simulink model "OFDM_Communication_Model_Start"  (R2024a)
settings: Solver=FixedStepDiscrete  StartTime=0.0  StopTime=0.2*4  RelTol=1e-3  EnableMultiTasking=on
model workspace: external: MAT-File modelspace.mat (data not in the file)
libraries: dspxfrm3 x3, commdigbbndpm3 x2, matrix_library x2
settings Model: Creator=thua3267  LastModifiedBy=hcha7553
settings SolverCC: AlgebraicLoopSolver=TrustRegion  AutoInsertRateTranBlk=on
settings DataIOCC: LimitDataPoints=on  ReturnWorkspaceOutputs=off
settings OptimizationCC: LifeSpan=inf
settings DebuggingCC: UnconnectedInputMsg=warning  UnconnectedOutputMsg=warning  UnconnectedLineMsg=warning  AllowSymbolicDim=off  SFUnexpectedBacktrackingDiag=warning  SFNoUnconditionalDefaultTransitionDiag=warning  SFExecutionAtInitializationDiag=none  ArithmeticOperatorsInVariantConditions=warning
settings ModelReferenceCC: EnableRefExpFcnMdlSchedulingChecks=on  PropagateSignalLabelsOutOfModel=off
settings SFSimCC: SimUseLocalCustomCode=off  CustomCodeUndefinedFunction=UseInterfaceOnly
settings RTWCC: RTWUseLocalCustomCode=off  GPUComputeCapability=3.5
settings CodeAppCC: StateflowObjectComments=on
settings GRTTargetCC: TargetLangStandard=C89/C90 (ANSI)
settings ConfigComp: CovMetricSettings=dw  CovSaveCumulativeToWorkspaceVar=on  CovSaveSingleToWorkspaceVar=on  CovExternalEMLEnable=off

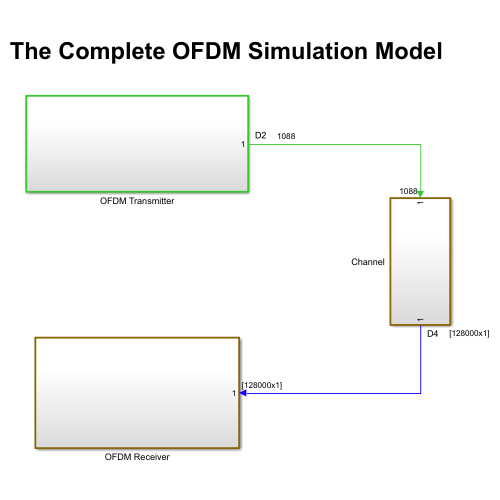
[thumbnail: Simulink's stored preview of the top-level diagram]
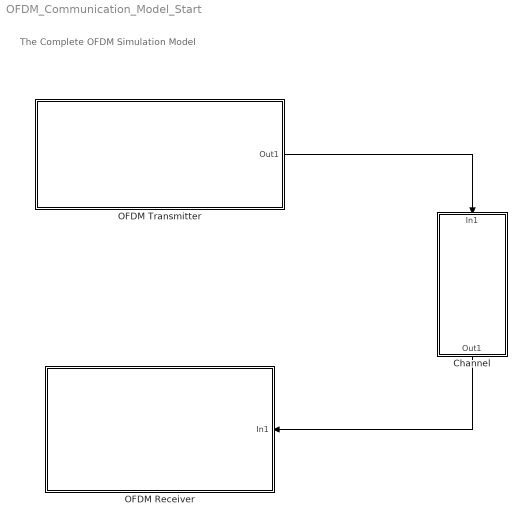
== system OFDM_Communication_Model_Start ==
  note: The Complete OFDM Simulation Model
  Channel : Subsystem
  OFDM Receiver : Subsystem
  OFDM Transmitter : Subsystem
  wires:
  OFDM Transmitter/1(Out1) -> Channel/1(In1)
  Channel/1(Out1) -> OFDM Receiver/1(In1)

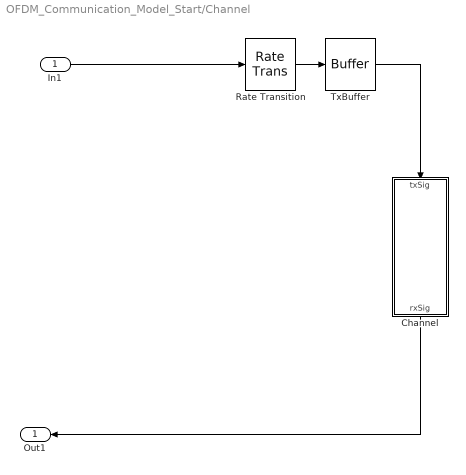
== system OFDM_Communication_Model_Start/Channel ==
  In1 : Inport
  Channel : MATLAB Function  TreatAsAtomicUnit=on
  Rate Transition : RateTransition  OutPortSampleTime=1/640e3*1280
  TxBuffer : Buffer  N=128000
  Out1 : Outport  VectorParamsAs1DForOutWhenUnconnected=off
  wires:
  In1/1 -> Rate Transition/1
  Channel/1(rxSig) -> Out1/1
  TxBuffer/1 -> Channel/1(txSig)
  Rate Transition/1 -> TxBuffer/1

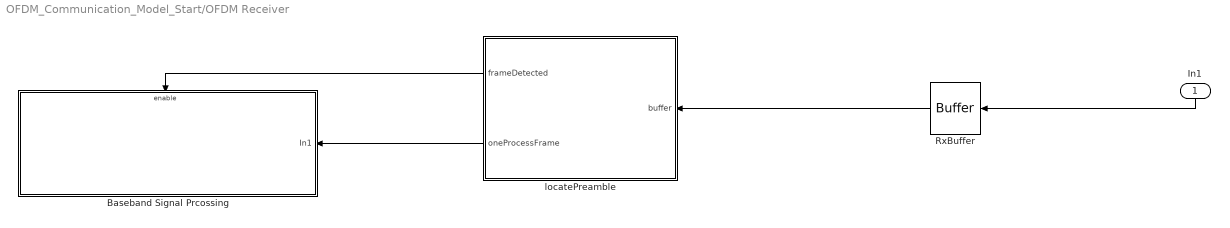
== system OFDM_Communication_Model_Start/OFDM Receiver ==
  In1 : Inport
  Baseband Signal Prcossing : Subsystem  TreatAsAtomicUnit=on
  RxBuffer : Buffer  N=1280*2  V=1280
  locatePreamble : MATLAB Function  TreatAsAtomicUnit=on
  wires:
  locatePreamble/2(oneProcessFrame) -> Baseband Signal Prcossing/1(In1)
  locatePreamble/1(frameDetected) -> Baseband Signal Prcossing/Enable
  In1/1 -> RxBuffer/1
  RxBuffer/1 -> locatePreamble/1(buffer)

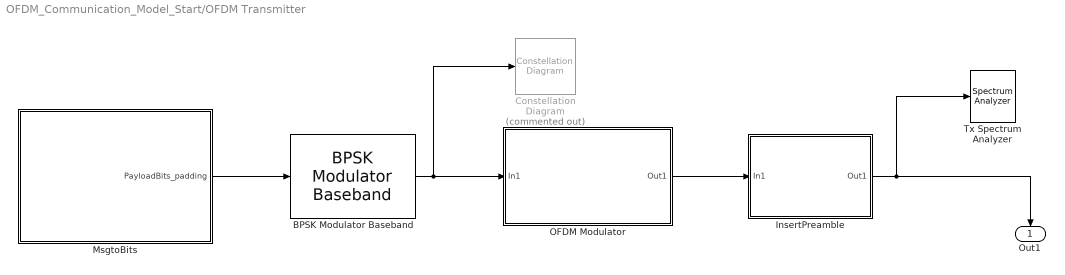
== system OFDM_Communication_Model_Start/OFDM Transmitter ==
  BPSK Modulator Baseband : commdigbbndpm3/BPSK Modulator Baseband  Ph=0  outDtype=double  outWordLen=16  outUDDataType=sfix(16)  outFracLenMode=Best precision  outFracLen=15  outDataTypeStr=double  outLastDataTypeStr=double
  Constellation Diagram : ConstellationDiagram  Commented=on  WindowPosition=[1 41 1920 964]  DefaultConfigurationName=comm.scopes.ConstellationDiagramBlockCfg
  InsertPreamble : Subsystem
  MsgtoBits : MATLAB Function  TreatAsAtomicUnit=on
  OFDM Modulator : Subsystem
  Tx Spectrum Analyzer : SpectrumAnalyzer  WindowPosition=[491.000000,211.000000,299.000000,298.000000,]  Visible=on  ScopeFrameLocation=window  Method=Welch  SampleRate=640000  Span=544000  StartFrequency=-272000  StopFrequency=272000  AveragingMethod=Running  YLimits=[-78.9896859,-0.36696175]  ColorLimits=[-29.698374910183748,-7.1171834026087382]  AllowFFTLengthLessThanSamplesPerUpdate=on  DefaultConfigurationName=spbscopes.SpectrumAnalyzerBlockCfg  IsFrequencyInputMode=0  FrequencyVectorPort=0  FrequencyVectorFromPort=0  FrequencyInputRBWPort=0  FrequencyInputRBWFromPort=0
  Out1 : Outport  VectorParamsAs1DForOutWhenUnconnected=off
  wires:
  MsgtoBits/1(PayloadBits_padding) -> BPSK Modulator Baseband/1
  InsertPreamble/1(Out1) -> Out1/1, Tx Spectrum Analyzer/1
  BPSK Modulator Baseband/1 -> Constellation Diagram/1, OFDM Modulator/1(In1)
  OFDM Modulator/1(Out1) -> InsertPreamble/1(In1)

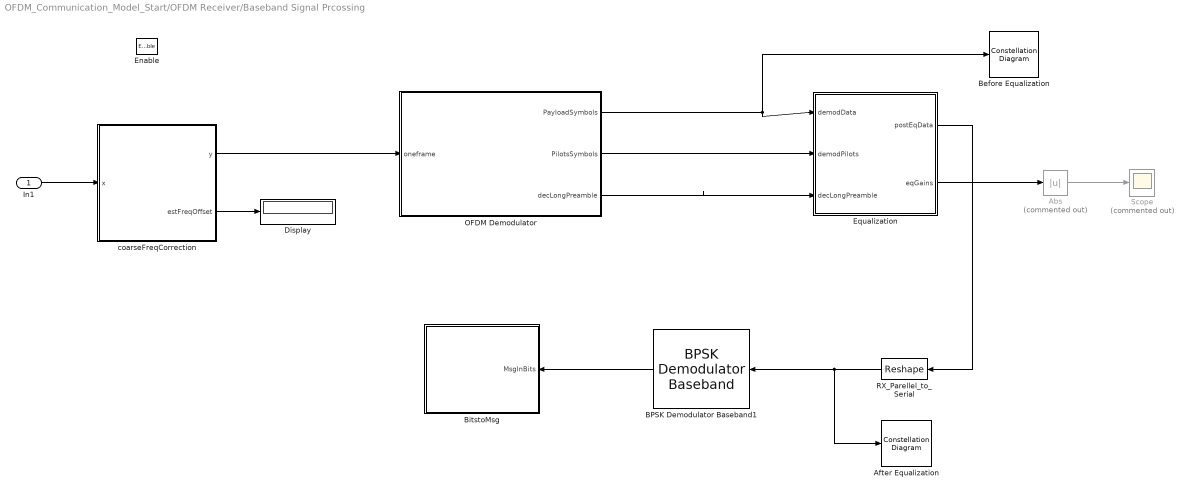
== system OFDM_Communication_Model_Start/OFDM Receiver/Baseband Signal Prcossing ==
  In1 : Inport
  Enable : EnablePort
  " Equalization" : MATLAB Function  TreatAsAtomicUnit=on
  " RX_Parellel_to_Serial" : Reshape  OutputDimensionality=Column vector (2-D)
  " coarseFreqCorrection" : MATLAB Function  TreatAsAtomicUnit=on
  Abs : Abs  Commented=on  SaturateOnIntegerOverflow=off
  After Equalization : ConstellationDiagram  WindowPosition=[486.000000,209.000000,309.000000,302.000000,]  Visible=on  ScopeFrameLocation=window  SymbolsToDisplay=12  ReferenceConstellation=BPSK  XLimits=[-4 4]  YLimits=[-4 4]  DefaultConfigurationName=comm.scopes.ConstellationDiagramBlockCfg
  BPSK Demodulator Baseband1 : commdigbbndpm3/BPSK Demodulator Baseband  DecType=Hard decision  VarSource=Dialog  Variance=1  Ph=0  outDtype=Inherit via internal rule  derotateFactorWordLen=16  derotateFactorDataTypeStr=Inherit: Same word length as input  derotateFactorLastDataTypeStr=Inherit: Same word length as input
  Before Equalization : ConstellationDiagram  WindowPosition=[474.000000,209.000000,332.000000,302.000000,]  Visible=on  ScopeFrameLocation=window  SymbolsToDisplay=1  ReferenceConstellation=BPSK  XLimits=[-0.039844 0.03808]  YLimits=[-0.043559 0.034365]  DefaultConfigurationName=comm.scopes.ConstellationDiagramBlockCfg
  BitstoMsg : MATLAB Function  TreatAsAtomicUnit=on
  Display : Display
  OFDM Demodulator : Subsystem
  Scope : Scope  Commented=on
  wires:
  In1/1 -> " coarseFreqCorrection"/1(x)
  " coarseFreqCorrection"/2(estFreqOffset) -> Display/1
  BPSK Demodulator Baseband1/1 -> BitstoMsg/1(MsgInBits)
  " Equalization"/1(postEqData) -> " RX_Parellel_to_Serial"/1
  " RX_Parellel_to_Serial"/1 -> After Equalization/1, BPSK Demodulator Baseband1/1
  " coarseFreqCorrection"/1(y) -> OFDM Demodulator/1(oneframe)
  " Equalization"/2(eqGains) -> Abs/1
  Abs/1 -> Scope/1
  OFDM Demodulator/1(PayloadSymbols) -> Before Equalization/1, " Equalization"/1(demodData)
  OFDM Demodulator/2(PilotsSymbols) -> " Equalization"/2(demodPilots)
  OFDM Demodulator/3(decLongPreamble) -> " Equalization"/3(decLongPreamble)

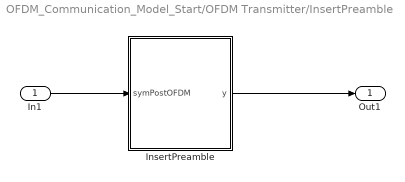
== system OFDM_Communication_Model_Start/OFDM Transmitter/InsertPreamble ==
  In1 : Inport
  InsertPreamble : MATLAB Function  TreatAsAtomicUnit=on
  Out1 : Outport  VectorParamsAs1DForOutWhenUnconnected=off
  wires:
  InsertPreamble/1(y) -> Out1/1
  In1/1 -> InsertPreamble/1(symPostOFDM)

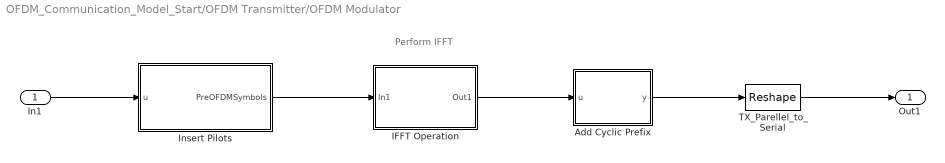
== system OFDM_Communication_Model_Start/OFDM Transmitter/OFDM Modulator ==
  note: Perform IFFT
  In1 : Inport
  " TX_Parellel_to_Serial" : Reshape  OutputDimensionality=Column vector (2-D)
  Add Cyclic Prefix : MATLAB Function  TreatAsAtomicUnit=on
  IFFT Operation : Subsystem
  Insert Pilots : MATLAB Function  TreatAsAtomicUnit=on
  Out1 : Outport  VectorParamsAs1DForOutWhenUnconnected=off
  wires:
  " TX_Parellel_to_Serial"/1 -> Out1/1
  Add Cyclic Prefix/1(y) -> " TX_Parellel_to_Serial"/1
  In1/1 -> Insert Pilots/1(u)
  Insert Pilots/1(PreOFDMSymbols) -> IFFT Operation/1(In1)
  IFFT Operation/1(Out1) -> Add Cyclic Prefix/1(u)

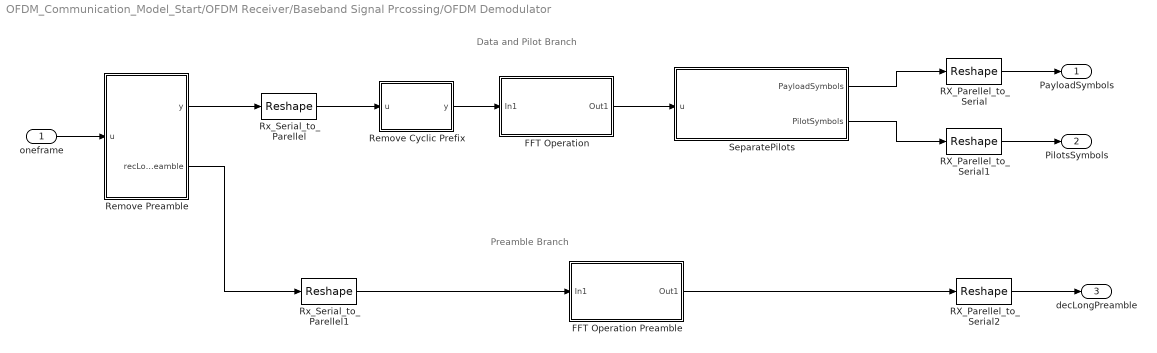
== system OFDM_Communication_Model_Start/OFDM Receiver/Baseband Signal Prcossing/OFDM Demodulator ==
  note: Data and Pilot Branch
  note: Preamble Branch
  oneframe : Inport
  " RX_Parellel_to_Serial" : Reshape  OutputDimensionality=Column vector (2-D)
  " RX_Parellel_to_Serial1" : Reshape  OutputDimensionality=Column vector (2-D)
  " RX_Parellel_to_Serial2" : Reshape  OutputDimensionality=Column vector (2-D)
  FFT Operation : Subsystem
  FFT Operation Preamble : Subsystem
  Remove Cyclic Prefix : MATLAB Function  TreatAsAtomicUnit=on
  "Remove Preamble " : MATLAB Function  TreatAsAtomicUnit=on
  Rx_Serial_to_Parellel : Reshape  OutputDimensionality=Customize  OutputDimensions=[80 12]
  Rx_Serial_to_Parellel1 : Reshape  OutputDimensionality=Customize  OutputDimensions=[64 2]
  SeparatePilots : MATLAB Function  TreatAsAtomicUnit=on
  PayloadSymbols : Outport  VectorParamsAs1DForOutWhenUnconnected=off
  PilotsSymbols : Outport  Port=2  VectorParamsAs1DForOutWhenUnconnected=off
  decLongPreamble : Outport  Port=3  VectorParamsAs1DForOutWhenUnconnected=off
  wires:
  " RX_Parellel_to_Serial"/1 -> PayloadSymbols/1
  Rx_Serial_to_Parellel/1 -> Remove Cyclic Prefix/1(u)
  Remove Cyclic Prefix/1(y) -> FFT Operation/1(In1)
  FFT Operation/1(Out1) -> SeparatePilots/1(u)
  SeparatePilots/1(PayloadSymbols) -> " RX_Parellel_to_Serial"/1
  "Remove Preamble "/1(y) -> Rx_Serial_to_Parellel/1
  oneframe/1 -> "Remove Preamble "/1(u)
  SeparatePilots/2(PilotSymbols) -> " RX_Parellel_to_Serial1"/1
  " RX_Parellel_to_Serial1"/1 -> PilotsSymbols/1
  FFT Operation Preamble/1(Out1) -> " RX_Parellel_to_Serial2"/1
  " RX_Parellel_to_Serial2"/1 -> decLongPreamble/1
  "Remove Preamble "/2(recLongPreamble) -> Rx_Serial_to_Parellel1/1
  Rx_Serial_to_Parellel1/1 -> FFT Operation Preamble/1(In1)

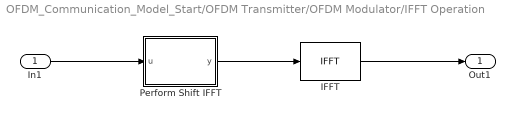
== system OFDM_Communication_Model_Start/OFDM Transmitter/OFDM Modulator/IFFT Operation ==
  In1 : Inport
  IFFT : dspxfrm3/IFFT  FFTImplementation=Auto  CompMethod=Table lookup  TableOpt=NEW  TableOptActive=Speed  BitRevOrder=off  cs_in=off  Normalize=on  InheritFFTLength=on  FFTLength=64  WrapInput=on  mode=Complex  outSamplingMode=Sample based  roundingMode=Floor  overflowMode=off  firstCoeffDataTypeStr=Inherit: Same word length as input  firstCoeffLastDataTypeStr=Inherit: Same word length as input  outputMin=[]  outputMax=[]
  Perform Shift IFFT : MATLAB Function  TreatAsAtomicUnit=on
  Out1 : Outport  VectorParamsAs1DForOutWhenUnconnected=off
  wires:
  IFFT/1 -> Out1/1
  In1/1 -> Perform Shift IFFT/1(u)
  Perform Shift IFFT/1(y) -> IFFT/1

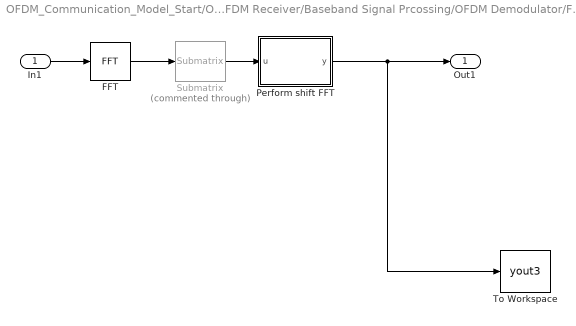
== system OFDM_Communication_Model_Start/OFDM Receiver/Baseband Signal Prcossing/OFDM Demodulator/FFT Operation ==
  In1 : Inport
  FFT : dspxfrm3/FFT  FFTImplementation=Auto  CompMethod=Table lookup  TableOpt=NEW  TableOptActive=Speed  BitRevOrder=off  Normalize=on  InheritFFTLength=on  FFTLength=64  WrapInput=on  roundingMode=Floor  overflowMode=off  firstCoeffDataTypeStr=Inherit: Same word length as input  firstCoeffLastDataTypeStr=Inherit: Same word length as input  outputMin=[]  outputMax=[]
  Perform shift FFT : MATLAB Function  TreatAsAtomicUnit=on
  Submatrix : matrix_library/Submatrix  Commented=through  RowSpan=Range of rows  RowStartMode=First  RowStartIndex=1  RowEndMode=Index  RowEndIndex=64  ColSpan=Range of columns  ColStartMode=First  ColStartIndex=1  ColEndMode=Last  ColEndIndex=1
  To Workspace : ToWorkspace  VariableName=yout3  SampleTime=-1
      settings: Save2DSignal=2-D array (concatenate along first dimension)
  Out1 : Outport  VectorParamsAs1DForOutWhenUnconnected=off
  wires:
  FFT/1 -> Submatrix/1
  In1/1 -> FFT/1
  Submatrix/1 -> Perform shift FFT/1(u)
  Perform shift FFT/1(y) -> To Workspace/1, Out1/1

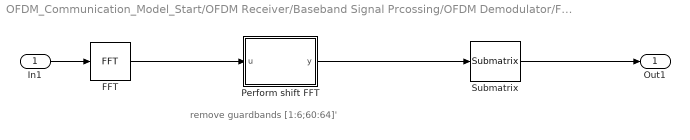
== system OFDM_Communication_Model_Start/OFDM Receiver/Baseband Signal Prcossing/OFDM Demodulator/FFT Operation Preamble ==
  note: remove guardbands [1:6;60:64]'
  In1 : Inport
  FFT : dspxfrm3/FFT  FFTImplementation=Auto  CompMethod=Table lookup  TableOpt=NEW  TableOptActive=Speed  BitRevOrder=off  Normalize=on  InheritFFTLength=on  FFTLength=64  WrapInput=on  roundingMode=Floor  overflowMode=off  firstCoeffDataTypeStr=Inherit: Same word length as input  firstCoeffLastDataTypeStr=Inherit: Same word length as input  outputMin=[]  outputMax=[]
  Perform shift FFT : MATLAB Function  TreatAsAtomicUnit=on
  Submatrix : matrix_library/Submatrix  RowSpan=Range of rows  RowStartMode=Index  RowStartIndex=7  RowEndMode=Index  RowEndIndex=59  ColSpan=All columns  ColStartMode=First  ColStartIndex=1  ColEndMode=Last  ColEndIndex=1
  Out1 : Outport  VectorParamsAs1DForOutWhenUnconnected=off
  wires:
  In1/1 -> FFT/1
  FFT/1 -> Perform shift FFT/1(u)
  Perform shift FFT/1(y) -> Submatrix/1
  Submatrix/1 -> Out1/1

== matlab function OFDM_Communication_Model_Start/OFDM Receiver/Baseband Signal Prcossing/OFDM Demodulator/Remove Preamble  ==
  data: u input; y output; recLongPreamble output
function [y, recLongPreamble] = rmPreamble(u)
%Separate data from preambles
%y data and pilot symbols

%%Configuration Parameters
FFTLen=64;

%% Alorithm 
y=u(5*FFTLen+1:end);
recLongPreamble=u(3*FFTLen + (1:2*FFTLen));

== matlab function OFDM_Communication_Model_Start/OFDM Receiver/Baseband Signal Prcossing/BitstoMsg ==
  data: MsgInBits input; NumFrameDetected data_store_memory; SystemBER data_store_memory
function BitstoMsg(MsgInBits)

% Configuration paramters
PayloadMessage = 'Welcome to the school of Electrical and Computer Engineering, Uni. of Sydney!';
NumBitsPerCharacter  = 7;
global NumFrameDetected;    %count the number of frame correctly received
global SystemBER;
coder.extrinsic('dec2bin','fprintf','num2str');
%% Alorithm

if NumFrameDetected < 100; %only display first 80 frame, avoid channel sample cut
    % transmitted message

    txMsgInBits    = coder.const(double(dec2bin(PayloadMessage, NumBitsPerCharacter).'));
    txMsgInBits    = txMsgInBits(:) - 48;
    bitMsgLen      = length(txMsgInBits);

    % received message
    %remove padding
    rxMsgInBits = MsgInBits(1:bitMsgLen,:);
    decMsgInBits = reshape(rxMsgInBits(1:bitMsgLen),[7, bitMsgLen/7])';
    fprintf('Received message:\n')
    disp(char(bin2dec(num2str(decMsgInBits)))');

    %% BER
    % BER calculation
    numBitErr = sum(txMsgInBits(:) ~= rxMsgInBits(:));
        BER = numBitErr/(bitMsgLen);
        SystemBER = (SystemBER*(NumFrameDetected-1) + BER)/NumFrameDetected;%accumulated BER
        fprintf('Error Stats:\nTotal number of Frame detected = %d.  The OFDM System average BER = %f\n\n', ...
             NumFrameDetected, SystemBER);
end

== matlab function OFDM_Communication_Model_Start/OFDM Receiver/Baseband Signal Prcossing/ Equalization ==
  data: demodData input; demodPilots input; postEqData output; FreqOffsetEstBuffer data_store_memory; NumFrameDetected data_store_memory; decLongPreamble input; eqGains output
function [postEqData, eqGains] = equalization(demodData, demodPilots, decLongPreamble)
 % Equalize the OFDM frame through the use of both the long preamble
% from the 802.11a standard and four pilot tones in the data frames.
% The gains from the pilots are interpolated across frequency and
% applied to all data subcarriers.

%% Configuration Parameters
% Use long preamble frame to estimate channel in frequency domain
NumOFDMSymbols=12;
NumDataCarriers=48;
NumPilotsCarriers=4;
NumGuardBandCarriers  = [6; 5];
PilotCarrierIndices   = [12;26;40;54];
DataCarrierIndices = [7:11,13:25,27:32,34:39,41:53,55:59]';%length=48, assuming DC at carrier 33  

%% Alogrithm
LongPreamble = complex(... 
        [ 1,  1, -1, -1,  1,  1, -1,  1, -1,  1,  1,  1,...
          1,  1,  1, -1, -1,  1,  1, -1,  1, -1,  1,  1,  1,  1, 0,...
          1, -1, -1,  1,  1, -1,  1, -1,  1, -1, -1, -1, -1, -1,...
          1,  1, -1, -1,  1, -1,  1, -1,  1,  1,  1,  1].', 0);

% Get preamble equalizer gains
preambleNorm = reshape(decLongPreamble,[53,2] )./ [LongPreamble, LongPreamble];
preambleEqGains = conj(mean(preambleNorm, 2)) ./ mean(abs(preambleNorm).^2, 2);    
              
% Calculate locations of pilots and data without guardbands in preambles
PilotIndexInPreamble = PilotCarrierIndices - NumGuardBandCarriers(1);
DataIndexInPreamble  = DataCarrierIndices - NumGuardBandCarriers(1);  
    
% Apply preamble equalizer gains to data and pilots
preambleEqGainsOnPilots = preambleEqGains(PilotIndexInPreamble);
preambleEqGainsOnData   = preambleEqGains(DataIndexInPreamble);
    
postEqPilots = repmat(preambleEqGainsOnPilots, [1, NumOFDMSymbols]) .* reshape(demodPilots, NumPilotsCarriers,NumOFDMSymbols);
postEqData   = repmat(preambleEqGainsOnData,   [1, NumOFDMSymbols]) .* reshape(demodData, NumDataCarriers,NumOFDMSymbols); 
    
% Get pilot equalizer gains
coder.extrinsic('getOFDMPreambleAndPilot_mymodel');
Pilots = coder.const(double(getOFDMPreambleAndPilot_mymodel('Pilot', NumOFDMSymbols)));
pilotNorm = postEqPilots ./ Pilots;
pilotEqGains = conj(pilotNorm) ./ (abs(pilotNorm).^2);
    
% Interpolate to data subcarrier size and apply pilot equalizer
% pilotEqGainsOnData = resample(pilotEqGains, NumDataCarriers/size(Pilots,
% 1), 1); Replace resample function with interp1
pilotEqGainsOnData = interp1(PilotCarrierIndices, pilotEqGains, DataCarrierIndices, 'pchip','extrap'); 
postEqData = pilotEqGainsOnData .* postEqData;
eqGains = [preambleEqGainsOnData, pilotEqGainsOnData];

% figure(7); plot(abs(pilotEqGainsOnData(:,4)));
figure(3); mesh(abs(pilotEqGainsOnData));
title('Equalization Gain');ylabel('Data subcarriers'),xlabel('OFDM symbols'),zlabel('Eq_Gain');

== matlab function OFDM_Communication_Model_Start/OFDM Receiver/Baseband Signal Prcossing/OFDM Demodulator/FFT Operation Preamble/Perform shift FFT ==
  data: u input; y output
function y = shiftFFT(u)
y=fftshift(u,1);

== matlab function OFDM_Communication_Model_Start/OFDM Transmitter/OFDM Modulator/Insert Pilots ==
  data: u input; PreOFDMSymbols output
function PreOFDMSymbols = InsertPilots(u)
%% Configuration paramters
%System Paramters
NumOFDMSymbols = 12;
NumDataCarriers = 48;%OFDM data carriers

%OFDM paramters 
FFTlen=64;
PilotCarrierIndices  = [12;26;40;54];%length=4
DataCarrierIndices = [7:11,13:25,27:32,34:39,41:53,55:59]';%length=48, assuming DC at carrier 33 
% GuardBandCarriers = [1:6, 60:64]'; %length=11
 
%% Algorithm
%Get pilot for each frame
coder.extrinsic('getOFDMPreambleAndPilot_mymodel');
Pilots = coder.const(double(getOFDMPreambleAndPilot_mymodel('Pilot', NumOFDMSymbols)));

%Reshape input payloaddata with padding 
ReshapedPayload= reshape(u,NumDataCarriers, NumOFDMSymbols);

%PreOFDMSymbols allocation
PreOFDMSymbols = complex(zeros(FFTlen, NumOFDMSymbols));
PreOFDMSymbols(PilotCarrierIndices,:) = Pilots;
PreOFDMSymbols(DataCarrierIndices ,:) = ReshapedPayload;

== matlab function OFDM_Communication_Model_Start/OFDM Transmitter/MsgtoBits ==
  data: PayloadBits_padding output
function PayloadBits_padding   = MsgtoBits
%This function converts a message to payloadBits with padding 

%% Configuration paramters
%System Paramters
   NumDataCarriers = 48;%OFDM data carriers
   NumBitsPerCharacter  = 7;
   BitsPerSymbol = 1; %bpsk 1,
   
%% Alogrithm 
%Payload message
    PayloadMessage = 'Welcome to the school of Electrical and Computer Engineering, Uni. of Sydney!';
    
%Convert message to bits
    coder.extrinsic('dec2bin');
    msgInBits = coder.const(double(dec2bin(PayloadMessage, NumBitsPerCharacter).'));
    PayloadBits = msgInBits(:) - 48;

% Calculate number of OFDM symbols per frame
   NumOFDMSymbols = ceil(length(PayloadBits)/BitsPerSymbol/NumDataCarriers);
   
% Calculate number of bits padded in each frame
   NumPadSymbols = NumDataCarriers * NumOFDMSymbols - length(PayloadBits)/BitsPerSymbol; %# of padded symbols required
   NumPadBits = NumPadSymbols * BitsPerSymbol; %# of padded bits required
    
%  PayloadBits with padding
    PayloadBits_padding = [PayloadBits; zeros(NumPadBits, 1)];

== matlab function OFDM_Communication_Model_Start/OFDM Transmitter/InsertPreamble/InsertPreamble ==
  data: y output; symPostOFDM input
function y = InsertPreamble(symPostOFDM)
%% Configuration paramters
FFTLength=64;
NumGuardBandCarriers = [6; 5];
NumFrames=1;

%% Alogrithm
%Get preamble for each frame
coder.extrinsic('getOFDMPreambleAndPilot_mymodel');
Preamble = coder.const(double(getOFDMPreambleAndPilot_mymodel('Preamble', FFTLength, NumGuardBandCarriers)));

% Repeat the frame
 y = repmat([Preamble; symPostOFDM], NumFrames, 1);%in general set NumFrames = 1. Let Block Buffer to repeat # of frames

== matlab function OFDM_Communication_Model_Start/OFDM Transmitter/OFDM Modulator/Add Cyclic Prefix ==
  data: u input; y output
function y = addCycPrefix(u)
%your code here
y=u;

== matlab function OFDM_Communication_Model_Start/Channel/Channel ==
  data: txSig input; rxSig output size=[128000, 1]
function rxSig = channel(txSig)
%% Configuraiton Parameters
%Adjustable channel parameters
EbN0dB = 25;            % Channel noise level (dB)
frequencyOffset = 5e5;  % Frequency offset (Hz)
phaseOffset = 15;       % Phase offset (Degrees)
delay = 80;             % Initial sample offset for entire data stream (samples)

s.sampleRate      = 640e3*1280;
s.FFTLength       = 64; 
s.numDataCarriers = 48;
s.CPLength        = 16;



%% Algorithm - Channel
% Pass signal through channel
rxSig = complex(zeros(128000,1));
coder.extrinsic('applyOFDMChannel_mymodel_20160225');
rxSig = applyOFDMChannel_mymodel_20160225(txSig, EbN0dB, delay, frequencyOffset, phaseOffset, s);

== matlab function OFDM_Communication_Model_Start/OFDM Transmitter/OFDM Modulator/IFFT Operation/Perform Shift IFFT ==
  data: u input; y output
function y = shiftIFFT(u)
y=ifftshift(u,1);

== matlab function OFDM_Communication_Model_Start/OFDM Receiver/locatePreamble ==
  data: buffer input; frameDetected output; oneProcessFrame output; NumFrameDetected data_store_memory
function [frameDetected,  oneProcessFrame] = locatePreamble(buffer)
%% Configuration Parameters
  FFTLength = 64;
  NumGuardBandCarriers=[6; 5];
  FrameLength=1280;
    
  %Modelspace Parameters
  global NumFrameDetected;
    
 %% Algorithm 
    % A few adjustable algorithms parameters:
    %   1). Number of frequency estimates to be averaged over for frequency corrections
    %    NumFreqToAverage=15;
    %   2). Peak threshold after normalization for preamble detection 
    PeakThreshold=0.6;
    %   3). Mininum number of peaks for positive match in frame detection
    MinNumPeaksForMatch=5;

    %pPreamble = coder.const(double(getOFDMPreambleAndPilot('Preamble', FFTLength, NumGuardBandCarriers)));
     pPreamble = (double(getOFDMPreambleAndPilot_mymodel('Preamble', FFTLength, NumGuardBandCarriers)));
     
    L = FFTLength;
    K = FFTLength/4; 
    known = pPreamble(1:K);
    windowLength = ceil(0.5*FrameLength + length(pPreamble));

    % Cross correlate
    rWin = buffer(1: windowLength-L+K-1);
    Phat = xcorr(rWin, conj(known));
    Rhat = xcorr(abs(rWin).^2, ones(K,1)); % Moving average

    % Remove leading and tail zeros overlaps
    PhatShort = Phat(ceil(length(Phat)/2):end-K/2+1);
    RhatShort = Rhat(ceil(length(Rhat)/2):end-K/2+1);

    % Calculate timing metric
    M = abs(PhatShort).^2 ./ RhatShort.^2;
    figure(2); plot(M);title('Locating Preamble');

    % Determine start of short preamble. First find peak locations
    MLocations = find(M > (max(M)*PeakThreshold));

    % Correct estimate to the start of preamble, not its center
    MLocations = MLocations - (K/2+1);
    
    % Determine correct peaks
    peaks = zeros(size(MLocations));
    desiredPeakLocations = (K:K:2*L)';
    for i = 1:length(MLocations)
        MLocationGuesses = MLocations(i) + desiredPeakLocations;
        peaks(i) = length(intersect(MLocations(i:end), MLocationGuesses));
    end

    % Have at least obj.pNumRequiredPeaks peaks for positive match    
    peaks(peaks < MinNumPeaksForMatch) = 0;

    % Pick earliest peak in time
    oneProcessFrame=complex(zeros(FrameLength,1)); 
    if ~isempty(peaks) 
        [numPeaks, frontPeakLocation] = max(peaks);
        if numPeaks > 0
             preambleStartLocation = MLocations(frontPeakLocation);
             %disp('check mate'); pause;
             oneProcessFrame = buffer(preambleStartLocation+(1:FrameLength));
             NumFrameDetected = NumFrameDetected+1;
        else 
            preambleStartLocation = -1; 
        end
    else % No desirable location found
        preambleStartLocation = -1;
    end
    
   frameDetected = (preambleStartLocation ~= -1 );

== matlab function OFDM_Communication_Model_Start/OFDM Receiver/Baseband Signal Prcossing/ coarseFreqCorrection ==
  data: x input; y output; estFreqOffset output; FreqOffsetEstBuffer data_store_memory; NumFrameDetected data_store_memory
function [y, estFreqOffset] = coarseFreqCorrection(x)
 % Frequency correction based on the Schmidl and Cox method, utilizing
 % halves of the short preamble from the 802.11a standard.
 
%% System parameters
 SampleRate = 640e3;
 FFTLength = 64;
 
 %Model space paramter
 global FreqOffsetEstBuffer; %buffer of size 15
 global NumFrameDetected;    %count the number of frame correctly received

 %% Alogrithm based on the Schmidl and Cox method   
 Ts = 1/SampleRate;
 halfFFTLen = FFTLength/2;
 freqOffsetBufferLen = 15;
    
 % Cross-correlate preamble and determine phase angle
 phi = angle(sum(conj(x(1:halfFFTLen)) .* x(halfFFTLen+(1:halfFFTLen)))); 
                     
 % Update frequency offset buffer
 bufferIdx = mod(NumFrameDetected - 1, freqOffsetBufferLen) + 1;
 FreqOffsetEstBuffer(bufferIdx) = phi/(2 * pi * halfFFTLen * Ts);
    
 % Estimated frequency offset     
 estFreqOffset = mean(FreqOffsetEstBuffer(1:min(freqOffsetBufferLen, NumFrameDetected)));
 
 % Apply frequency correction
 y = exp(1i * estFreqOffset * (0 : (length(x)-1))' * Ts) .* x;

end

== matlab function OFDM_Communication_Model_Start/OFDM Receiver/Baseband Signal Prcossing/OFDM Demodulator/FFT Operation/Perform shift FFT ==
  data: u input; y output
function y = shiftFFT(u)
y=fftshift(u,1);

== matlab function OFDM_Communication_Model_Start/OFDM Receiver/Baseband Signal Prcossing/OFDM Demodulator/Remove Cyclic Prefix ==
  data: u input; y output
function y = rmCycPref(u)
%your code here
y=u;

== matlab function OFDM_Communication_Model_Start/OFDM Receiver/Baseband Signal Prcossing/OFDM Demodulator/SeparatePilots ==
  data: u input; PayloadSymbols output; PilotSymbols output
function [PayloadSymbols, PilotSymbols] = SeparatePilots(u)
%% Configuration Parameter
DataCarrierIndices = [7:11,13:25,27:32,34:39,41:53,55:59]';%length=48, assuming DC at carrier 33 
PilotCarrierIndices  = [12;26;40;54];%length=4

%% Algorithm
%extract PayloadSymbols from each frame
PayloadSymbols = u(DataCarrierIndices,:);
PilotSymbols = u(PilotCarrierIndices,:);
